simulink model "microgrid_case5"  (R2026a)
settings: Solver=ode14x  FixedStep=50e-6
libraries: ee_lib x65, nesl_utility x33, fl_lib x29, simulink x2
(part 2 of 2)

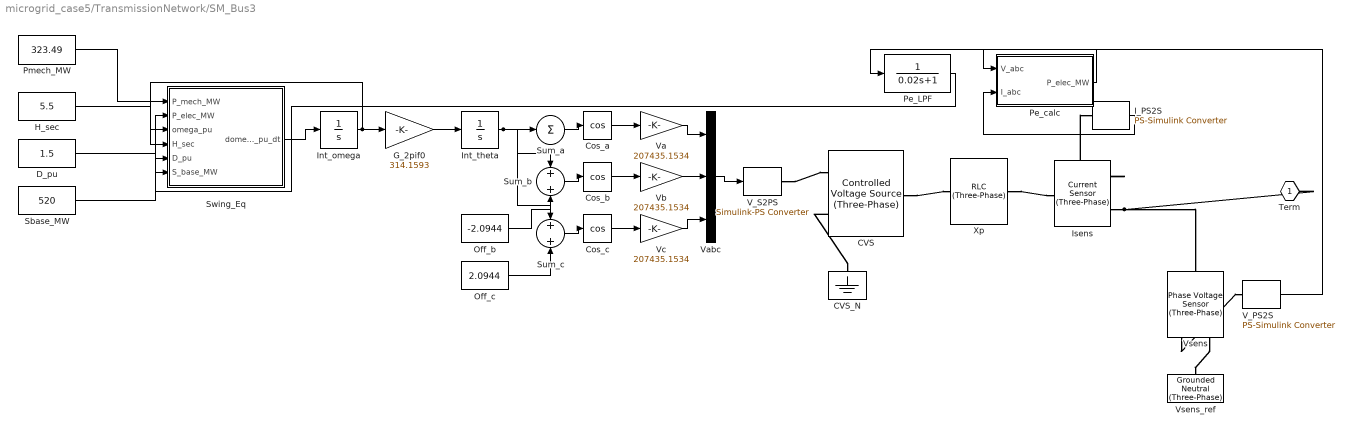
== system microgrid_case5/TransmissionNetwork/SM_Bus3 ==
  CVS : ee_lib/Sources/Controlled Voltage Source (Three-Phase)  input_option=ee.enum.inputType.instantaneous  FRated=60 Hz
  CVS_N : fl_lib/Electrical/Electrical Elements/Electrical Reference
  Cos_a : Trigonometry  Operator=cos
  Cos_b : Trigonometry  Operator=cos
  Cos_c : Trigonometry  Operator=cos
  D_pu : Constant  Value=1.5
  G_2pif0 : Gain  Gain=314.1593
  H_sec : Constant  Value=5.5
  I_PS2S : nesl_utility/PS-Simulink Converter  PhysicalDomain=network_engine_domain  SubClassName=ps_output  LeftPortType=input  RightPortType=output  PseudoPeriodic=off  Frequencies=[]  VectorFormat=inherit  Unit=inherit  AffineConversion=off
  Int_omega : Integrator  InitialCondition=1.0
  Int_theta : Integrator  InitialCondition=0.13268
  Isens : ee_lib/Sensors & Transducers/Current Sensor (Three-Phase)  port_option=ee.enum.threePhasePort.composite
  Off_b : Constant  Value=-2.0944
  Off_c : Constant  Value=2.0944
  Pe_LPF : TransferFcn  Denominator=[0.02 1]
  Pe_calc : MATLAB Function  TreatAsAtomicUnit=on
  Pmech_MW : Constant  Value=323.49
  Sbase_MW : Constant  Value=520
  Sum_a : Sum  Inputs=+
  Sum_b : Sum
  Sum_c : Sum
  Swing_Eq : MATLAB Function  TreatAsAtomicUnit=on
  V_PS2S : nesl_utility/PS-Simulink Converter  PhysicalDomain=network_engine_domain  SubClassName=ps_output  LeftPortType=input  RightPortType=output  PseudoPeriodic=off  Frequencies=[]  VectorFormat=inherit  Unit=inherit  AffineConversion=off
  V_S2PS : nesl_utility/Simulink-PS Converter  PhysicalDomain=network_engine_domain  SubClassName=ps_input  LeftPortType=input  RightPortType=output  PseudoPeriodic=off  Frequencies=[]  NoiseDistribution=none  NoiseParameters=[]  Unit=V  AffineConversion=off  FilteringAndDerivatives=filter  SimscapeFilterOrder=1  InputFilterTimeConstant=1e-4  UdotUserProvided=0
  Va : Gain  Gain=207435.1534
  Vabc : Mux  Inputs=3
  Vb : Gain  Gain=207435.1534
  Vc : Gain  Gain=207435.1534
  Vsens : ee_lib/Sensors & Transducers/Phase Voltage Sensor (Three-Phase)  port_option=ee.enum.threePhasePort.composite
  Vsens_ref : ee_lib/Connectors & References/Grounded Neutral (Three-Phase)  port_option=ee.enum.threePhasePort.composite
  Xp : ee_lib/Passive/RLC Assemblies/RLC (Three-Phase)  port_option=ee.enum.threePhasePort.composite  component_structure=ee.enum.rlc.structure.SeriesRL  R=0.001 Ohm  L=0.080955 H  C=1e-6 F  R_parasitic=0 Ohm  G_parasitic=0 1/Ohm  IL_specify=off  IL_priority=High  IL=[0, 0, 0] A  IL_nominal_specify=off  IL_nominal_value=1  IL_nominal_unit=A  VC_specify=off  VC_priority=High  VC=[0, 0, 0] V  VC_nominal_specify=off  VC_nominal_value=1  VC_nominal_unit=V
  Term : PMIOPort  Side=Right
  wires:
  V_PS2S/1 -> Pe_calc/1(V_abc)
  I_PS2S/1 -> Pe_calc/2(I_abc)
  Pe_calc/1(P_elec_MW) -> Pe_LPF/1
  Pmech_MW/1 -> Swing_Eq/1(P_mech_MW)
  Pe_LPF/1 -> Swing_Eq/2(P_elec_MW)
  Int_omega/1 -> Swing_Eq/3(omega_pu), G_2pif0/1
  H_sec/1 -> Swing_Eq/4(H_sec)
  D_pu/1 -> Swing_Eq/5(D_pu)
  Sbase_MW/1 -> Swing_Eq/6(S_base_MW)
  Swing_Eq/1(domega_pu_dt) -> Int_omega/1
  G_2pif0/1 -> Int_theta/1
  Int_theta/1 -> Sum_a/1, Sum_b/1, Sum_c/1
  Off_b/1 -> Sum_b/2
  Off_c/1 -> Sum_c/2
  Sum_a/1 -> Cos_a/1
  Sum_b/1 -> Cos_b/1
  Sum_c/1 -> Cos_c/1
  Cos_a/1 -> Va/1
  Cos_b/1 -> Vb/1
  Cos_c/1 -> Vc/1
  Va/1 -> Vabc/1
  Vb/1 -> Vabc/2
  Vc/1 -> Vabc/3
  Vabc/1 -> V_S2PS/1
  connections:
  CVS/LConn2 -- CVS_N/LConn1
  V_S2PS/RConn1 -- CVS/LConn1
  CVS/RConn1 -- Xp/LConn1
  Xp/RConn1 -- Isens/LConn1
  Term/RConn1 -- Isens/RConn2 -- Vsens/LConn1
  Vsens/RConn2 -- Vsens_ref/LConn1
  Isens/RConn1 -- I_PS2S/LConn1
  Vsens/RConn1 -- V_PS2S/LConn1

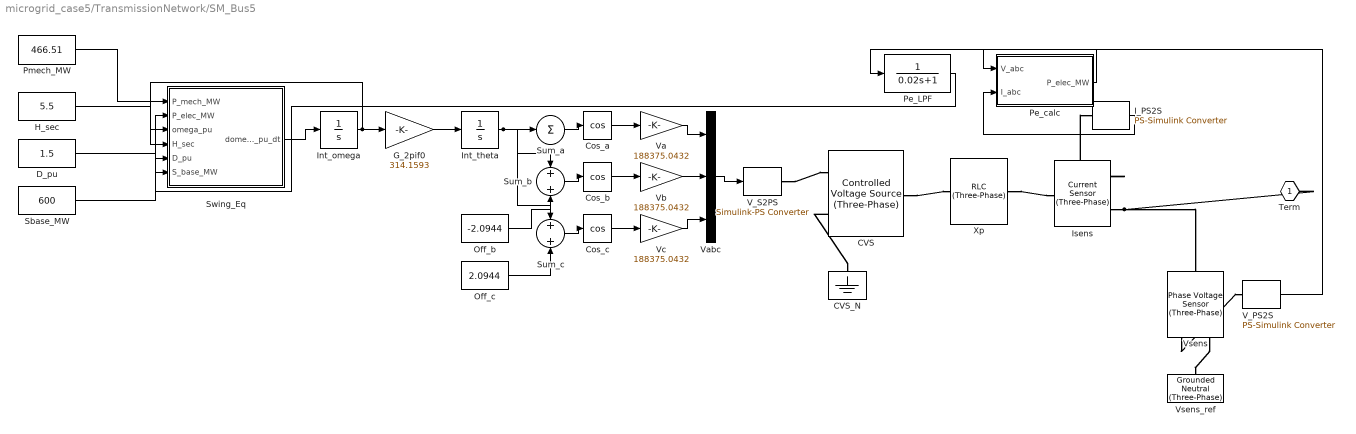
== system microgrid_case5/TransmissionNetwork/SM_Bus5 ==
  CVS : ee_lib/Sources/Controlled Voltage Source (Three-Phase)  input_option=ee.enum.inputType.instantaneous  FRated=60 Hz
  CVS_N : fl_lib/Electrical/Electrical Elements/Electrical Reference
  Cos_a : Trigonometry  Operator=cos
  Cos_b : Trigonometry  Operator=cos
  Cos_c : Trigonometry  Operator=cos
  D_pu : Constant  Value=1.5
  G_2pif0 : Gain  Gain=314.1593
  H_sec : Constant  Value=5.5
  I_PS2S : nesl_utility/PS-Simulink Converter  PhysicalDomain=network_engine_domain  SubClassName=ps_output  LeftPortType=input  RightPortType=output  PseudoPeriodic=off  Frequencies=[]  VectorFormat=inherit  Unit=inherit  AffineConversion=off
  Int_omega : Integrator  InitialCondition=1.0
  Int_theta : Integrator  InitialCondition=0.26678
  Isens : ee_lib/Sensors & Transducers/Current Sensor (Three-Phase)  port_option=ee.enum.threePhasePort.composite
  Off_b : Constant  Value=-2.0944
  Off_c : Constant  Value=2.0944
  Pe_LPF : TransferFcn  Denominator=[0.02 1]
  Pe_calc : MATLAB Function  TreatAsAtomicUnit=on
  Pmech_MW : Constant  Value=466.51
  Sbase_MW : Constant  Value=600
  Sum_a : Sum  Inputs=+
  Sum_b : Sum
  Sum_c : Sum
  Swing_Eq : MATLAB Function  TreatAsAtomicUnit=on
  V_PS2S : nesl_utility/PS-Simulink Converter  PhysicalDomain=network_engine_domain  SubClassName=ps_output  LeftPortType=input  RightPortType=output  PseudoPeriodic=off  Frequencies=[]  VectorFormat=inherit  Unit=inherit  AffineConversion=off
  V_S2PS : nesl_utility/Simulink-PS Converter  PhysicalDomain=network_engine_domain  SubClassName=ps_input  LeftPortType=input  RightPortType=output  PseudoPeriodic=off  Frequencies=[]  NoiseDistribution=none  NoiseParameters=[]  Unit=V  AffineConversion=off  FilteringAndDerivatives=filter  SimscapeFilterOrder=1  InputFilterTimeConstant=1e-4  UdotUserProvided=0
  Va : Gain  Gain=188375.0432
  Vabc : Mux  Inputs=3
  Vb : Gain  Gain=188375.0432
  Vc : Gain  Gain=188375.0432
  Vsens : ee_lib/Sensors & Transducers/Phase Voltage Sensor (Three-Phase)  port_option=ee.enum.threePhasePort.composite
  Vsens_ref : ee_lib/Connectors & References/Grounded Neutral (Three-Phase)  port_option=ee.enum.threePhasePort.composite
  Xp : ee_lib/Passive/RLC Assemblies/RLC (Three-Phase)  port_option=ee.enum.threePhasePort.composite  component_structure=ee.enum.rlc.structure.SeriesRL  R=0.001 Ohm  L=0.070161 H  C=1e-6 F  R_parasitic=0 Ohm  G_parasitic=0 1/Ohm  IL_specify=off  IL_priority=High  IL=[0, 0, 0] A  IL_nominal_specify=off  IL_nominal_value=1  IL_nominal_unit=A  VC_specify=off  VC_priority=High  VC=[0, 0, 0] V  VC_nominal_specify=off  VC_nominal_value=1  VC_nominal_unit=V
  Term : PMIOPort  Side=Right
  wires:
  V_PS2S/1 -> Pe_calc/1(V_abc)
  I_PS2S/1 -> Pe_calc/2(I_abc)
  Pe_calc/1(P_elec_MW) -> Pe_LPF/1
  Pmech_MW/1 -> Swing_Eq/1(P_mech_MW)
  Pe_LPF/1 -> Swing_Eq/2(P_elec_MW)
  Int_omega/1 -> Swing_Eq/3(omega_pu), G_2pif0/1
  H_sec/1 -> Swing_Eq/4(H_sec)
  D_pu/1 -> Swing_Eq/5(D_pu)
  Sbase_MW/1 -> Swing_Eq/6(S_base_MW)
  Swing_Eq/1(domega_pu_dt) -> Int_omega/1
  G_2pif0/1 -> Int_theta/1
  Int_theta/1 -> Sum_a/1, Sum_b/1, Sum_c/1
  Off_b/1 -> Sum_b/2
  Off_c/1 -> Sum_c/2
  Sum_a/1 -> Cos_a/1
  Sum_b/1 -> Cos_b/1
  Sum_c/1 -> Cos_c/1
  Cos_a/1 -> Va/1
  Cos_b/1 -> Vb/1
  Cos_c/1 -> Vc/1
  Va/1 -> Vabc/1
  Vb/1 -> Vabc/2
  Vc/1 -> Vabc/3
  Vabc/1 -> V_S2PS/1
  connections:
  CVS/LConn2 -- CVS_N/LConn1
  V_S2PS/RConn1 -- CVS/LConn1
  CVS/RConn1 -- Xp/LConn1
  Xp/RConn1 -- Isens/LConn1
  Term/RConn1 -- Isens/RConn2 -- Vsens/LConn1
  Vsens/RConn2 -- Vsens_ref/LConn1
  Isens/RConn1 -- I_PS2S/LConn1
  Vsens/RConn1 -- V_PS2S/LConn1

== matlab function microgrid_case5/TransmissionNetwork/SM_Bus5/Pe_calc ==
  data: V_abc input; P_elec_MW output; I_abc input
function P_elec_MW = Pe_calc(V_abc, I_abc)
%#codegen
% Instantaneous 3-phase electrical power at the machine terminal [MW].
    P_W       = V_abc(1)*I_abc(1) + V_abc(2)*I_abc(2) + V_abc(3)*I_abc(3);
    P_elec_MW = P_W / 1e6;
end

== matlab function microgrid_case5/PCC/PLL_freq ==
  settings: updateMethod=DISCRETE  sampleTime=5e-05
  data: v_abc input; f_meas_Hz output; dt_s input; f0_Hz input; Kp input; Ki input
function f_meas_Hz = PLL_freq(v_abc, dt_s, f0_Hz, Kp, Ki)
%#codegen
% Synchronous-reference-frame PLL on the MV phase voltages.
% Clarke (amplitude-invariant) → normalise → q-axis error → PI → θ.
% Persistent θ and integral are discrete states (HIL/codegen friendly).
    persistent th vi
    if isempty(th), th = 0; vi = 0; end
    va = v_abc(1); vb = v_abc(2); vc = v_abc(3);
    valpha = (2/3)*(va - 0.5*vb - 0.5*vc);
    vbeta  = (1/sqrt(3))*(vb - vc);
    Vm = hypot(valpha, vbeta) + 1e-9;       % avoid /0 at start-up
    sa = valpha/Vm; sb = vbeta/Vm;          % unit phasor (amplitude-independent)
    vq = -sa*sin(th) + sb*cos(th);          % q-axis error → 0 when locked
    vi = vi + Ki*vq*dt_s;                    % PI integral
    w  = 2*pi*f0_Hz + Kp*vq + vi;            % estimated angular frequency
    th = mod(th + w*dt_s, 2*pi);             % advance & wrap phase
    f_meas_Hz = w/(2*pi);
end

== matlab function microgrid_case5/PCC/V_to_pu ==
  data: v_abc input; V_pcc_pu output; Vbase_LL input
function V_pcc_pu = V_to_pu(v_abc, Vbase_LL)
%#codegen
% Line-to-line RMS per-unit from instantaneous phase voltages.
% Amplitude-invariant Clarke magnitude = peak phase amplitude;
% LL_RMS = peak_phase * sqrt(3)/sqrt(2)  →  pu = LL_RMS / Vbase_LL.
    va = v_abc(1); vb = v_abc(2); vc = v_abc(3);
    valpha = (2/3)*(va - 0.5*vb - 0.5*vc);
    vbeta  = (1/sqrt(3))*(vb - vc);
    Vphase_peak = hypot(valpha, vbeta);
    V_pcc_pu = Vphase_peak * sqrt(3/2) / Vbase_LL;
end

== matlab function microgrid_case5/PCC/PQ_calc ==
  data: v_abc input; P_MW output; i_abc input; Q_MVAr output
function [P_MW, Q_MVAr] = PQ_calc(v_abc, i_abc)
%#codegen
% Instantaneous three-phase active & reactive power at the MV node.
% Amplitude-invariant Clarke → P = 1.5(vα iα + vβ iβ),  Q = 1.5(vβ iα − vα iβ).
% Sign: + current is transmission→MG, so +P = MG importing (§1.1).
    va = v_abc(1); vb = v_abc(2); vc = v_abc(3);
    ia = i_abc(1); ib = i_abc(2); ic = i_abc(3);
    valpha = (2/3)*(va - 0.5*vb - 0.5*vc);  vbeta = (1/sqrt(3))*(vb - vc);
    ialpha = (2/3)*(ia - 0.5*ib - 0.5*ic);  ibeta = (1/sqrt(3))*(ib - ic);
    P_W   = 1.5*(valpha*ialpha + vbeta*ibeta);
    Q_VAR = 1.5*(vbeta*ialpha - valpha*ibeta);
    P_MW   = P_W   / 1e6;
    Q_MVAr = Q_VAR / 1e6;
end

== matlab function microgrid_case5/GridFormingVSC/vf_droop ==
  settings: updateMethod=DISCRETE  sampleTime=5e-05
  data: v_abc input; m_abc output; i_abc input; V_dc_V input; f_meas_Hz input; V_meas_pu input; V_ref_pu input; f_ref_Hz input; mode input; dt_s input; f0_Hz input; CB_grid input; f_cmd_Hz output; P_vsc_MW output; Q_vsc_MVAr output; cb_open output; i_d_A output; i_q_A output; i_d_ref_A output; i_q_ref_A output
function [m_abc, f_cmd_Hz, P_vsc_MW, Q_vsc_MVAr, cb_open, i_d_A, i_q_A, i_d_ref_A, i_q_ref_A] = vf_droop(v_abc, i_abc, V_dc_V, f_meas_Hz, V_meas_pu, V_ref_pu, f_ref_Hz, mode, dt_s, f0_Hz, CB_grid)
%#codegen
% Grid-forming V-f droop + A8 secondary restoration (IO_CONTRACTS §3.5).
% FAZ 1+2 (2026-07-04, G10): optional inner dq current loop, gated by
% inner_en below. Default inner_en=0 reproduces the legacy open-loop m
% synthesis EXACTLY (bit-for-bit bypass).
% Persistent discrete states: oscillator phase, P/Q filters, secondary
% integrators, soft-start clock, saturation flag, inner current-loop PIs.
S_base_VA = 350000000;    % droop power base = VSC rating
R_p   = 0.05;  R_q   = 0.05;   % droop SLOPES (G4: §3.5 "(1/R)" read as slope)
tauPQ = 0.01;                  % P/Q LPF [s] (G5)
Kp_f  = 0.1;  Ki_f  = 0.5;  df_max = 2.5;  % A8 f-restore + clamp
Kp_V  = 0.5;  Ki_V  = 2;  dV_max = 0.1;  % A8 V-restore + clamp
Vph_pk = 563.383;  Vdc_nom = 1500;  m_lim = 1;
t_soft = 0.2;                 % amplitude ramp [s] (G3)
t_blend = 0.1;                % post-close amplitude blend [s] (G8)
Kdc_WpV = 3.33333e+06;  P_exp_max_W = 1e+08;  % DC-link export droop (A)
Kp_i = 3.11143;  Ki_i = 39.0994;  % FAZ1+2 inner current PI (33kV side, G10)
L_c = 0.000990398;  R_c = 0.0124457;  % coupling L[H]/R[Ohm] = XFMR leakage (G1), no separate filter
n_t = 47.8261;  % step-up XFMR turns ratio MV/LV (G10a init fix): AVVSC=LV, sensing=MV
i_max_pk = 9525.79;  % current limit, PEAK amps (id/iq are peak-scale, amplitude-invariant)
ilim_exit = 0.95*i_max_pk;  t_ib = 0.005;  % FAZ3 (G10b) limit hysteresis-lo + exit blend [s]
inner_en = 1;  % FAZ3 enable: 0=pure legacy voltage-forming, 1=overcurrent current-limiter armed
    persistent th P_f Q_f int_f int_V t_run sat_prev cb_state t_close id_int iq_int inner_prev ilim_on w_blend
    if isempty(th)
        % G8: start the LV oscillator ON the measured bus phase so the
        % pre-sync pull converges fast (Yg/D11: MV leads LV +30°).
        th = atan2((1/sqrt(3))*(v_abc(2)-v_abc(3)), ...
                   (2/3)*(v_abc(1)-0.5*v_abc(2)-0.5*v_abc(3))) - pi/6;
        P_f=0; Q_f=0; int_f=0; int_V=0; t_run=0; sat_prev=0;
        cb_state=0; t_close=0;              % G8: sync breaker starts OPEN
        id_int=0; iq_int=0; inner_prev=0;   % FAZ1+2: inner current-loop PI states + edge flag (G10a)
        ilim_on=0; w_blend=0;               % FAZ3 (G10b): overcurrent latch + legacy<->inner blend weight
    end

    % ── Instantaneous P/Q at the 33 kV terminal (amplitude-invariant Clarke)
    va=v_abc(1); vb=v_abc(2); vc=v_abc(3); ia=i_abc(1); ib=i_abc(2); ic=i_abc(3);
    valpha=(2/3)*(va-0.5*vb-0.5*vc);  vbeta=(1/sqrt(3))*(vb-vc);
    ialpha=(2/3)*(ia-0.5*ib-0.5*ic);  ibeta=(1/sqrt(3))*(ib-ic);
    P_W   = 1.5*(valpha*ialpha + vbeta*ibeta);   % + = injecting into AC bus
    Q_VAR = 1.5*(vbeta*ialpha - valpha*ibeta);
    P_f = P_f + (P_W   - P_f)*dt_s/tauPQ;        % 1st-order measurement LPF
    Q_f = Q_f + (Q_VAR - Q_f)*dt_s/tauPQ;
    Vdc_eff = max(V_dc_V, 0.5*Vdc_nom);          % FAZ1+2: moved up, needed before the oscillator section

    % ── Soft-start amplitude ramp (G3); integrators frozen until the
    % sync breaker is closed AND the post-close blend is done (G8).
    t_run = t_run + dt_s;
    soft  = min(t_run/t_soft, 1);
    conn  = (cb_state > 0.5) && (t_run - t_close >= t_blend);

    if mode > 0.5   % ─── GRID-FORMING (A2: no anti-islanding delay) ───
        % A8 secondary restoration: slow PIs trim f_ref/V_ref so the
        % steady state returns to the setpoints despite the droop offset.
        err_f = f_ref_Hz - f_meas_Hz;
        err_V = V_ref_pu - V_meas_pu;
        % Rule 7 anti-windup: integrate only when the modulator was NOT
        % saturated last step and the unit is CONNECTED + blended (G8).
        if sat_prev < 0.5 && conn
            int_f = int_f + Ki_f*err_f*dt_s;
            int_V = int_V + Ki_V*err_V*dt_s;
        end
        int_f = max(-df_max, min(df_max, int_f));    % clamp (Rule 7)
        int_V = max(-dV_max, min(dV_max, int_V));
        df_restore = max(-df_max, min(df_max, Kp_f*err_f + int_f));
        dV_restore = max(-dV_max, min(dV_max, Kp_V*err_V + int_V));

        % DC-LINK VOLTAGE DROOP (A): export DC-bus surplus to the grid. When
        % V_dc rises above nominal (ESS saturated on surplus renewables), bias
        % the droop frequency UP so the VSC angle leads the grid and real power
        % flows OUT, pulling V_dc back. df_export = R_p*f0*(P_export/S) makes the
        % converter settle at P=P_export (steady state f_cmd=grid f). Grid-
        % connected ONLY (CB_grid) AND synced (conn); island has no grid → 0.
        df_export = 0;
        if CB_grid > 0.5 && conn
            P_exp_W = Kdc_WpV*(V_dc_V - Vdc_nom);
            if P_exp_W < 0, P_exp_W = 0; end
            if P_exp_W > P_exp_max_W, P_exp_W = P_exp_max_W; end
            df_export = R_p*f0_Hz*(P_exp_W/S_base_VA);
        end
        % PRIMARY droop (slope form, G4): rated P → R_p·f0 Hz sag.
        f_cmd_Hz = (f_ref_Hz + df_restore + df_export) - R_p*(P_f/S_base_VA)*f0_Hz;
        V_cmd_pu = (V_ref_pu + dV_restore) - R_q*(Q_f/S_base_VA);
    else            % ─── GRID-FOLLOWING (stub, G7) ───
        f_cmd_Hz = f_meas_Hz;        % track the grid; droop/secondary off
        V_cmd_pu = V_ref_pu;
    end

    % ══════════════════════════════════════════════════════════════════
    % FAZ 1+2 (G10) — INNER dq CURRENT LOOP, island/grid-forming path only.
    % Yazdani & Iravani 2010 cascaded VSC control. th used below is THIS
    % sample angle (BEFORE the oscillator update further down) — the same
    % instant the v_abc/i_abc measurements were taken.
    % ══════════════════════════════════════════════════════════════════
    c_th = cos(th); s_th = sin(th);
    i_d_A = ialpha*c_th + ibeta*s_th;   % Park (amplitude-invariant -> PEAK
    i_q_A = -ialpha*s_th + ibeta*c_th;  % scale, matches i_abc directly, NOT rms)
    % ══ FAZ 3 (G10b): GRID-FORMING with CURRENT LIMITING (Rocabert 2012). The
    % VSC stays VOLTAGE-forming (m_abc_legacy forms f) in NORMAL operation; the
    % inner dq loop engages ONLY on OVERCURRENT, as a current LIMITER. It is NOT
    % an always-on current source (that let nobody form f -> f drifted to 53.76
    % Hz). Hysteresis latch: enter at i_max, leave below ilim_exit (0.95*i_max).
    i_mag = sqrt(i_d_A*i_d_A + i_q_A*i_q_A);
    if i_mag > i_max_pk,  ilim_on = 1; end   % over-limit -> arm the limiter
    if i_mag < ilim_exit, ilim_on = 0; end   % recovered  -> release (hysteresis)
    inner_active = double((mode > 0.5) && (inner_en > 0.5) && conn && (ilim_on > 0.5));
    % Output blend weight w_blend: jumps to 1 while limiting (the G10a bumpless
    % preload keeps the ENTRY step-free), decays to 0 over t_ib on release (soft
    % handback to legacy voltage-forming). inner_compute keeps the inner PI/phasor
    % coherent through the decay window so the blend has a live target.
    if inner_active > 0.5
        w_blend = 1;
    else
        w_blend = max(0, w_blend - dt_s/t_ib);
    end
    inner_compute = (inner_active > 0.5) || (w_blend > 1e-3);
    if inner_compute
        v_d = valpha*c_th + vbeta*s_th;
        v_q = -valpha*s_th + vbeta*c_th;
        % FAZ 3 current reference = the MEASURED current direction clamped onto
        % the i_max_pk circle. Over-limit: scl<1 pulls |i| down to i_max (id/iq
        % share preserved -- the protective action). Blend-out (not over-limit):
        % scl=1 = identity -> the inner voltage tracks the present operating
        % point and converges to legacy, so the handback is smooth.
        if inner_active > 0.5 && i_mag > 1e-6
            scl = i_max_pk / i_mag;
        else
            scl = 1;
        end
        i_d_ref_A = i_d_A * scl;
        i_q_ref_A = i_q_A * scl;
        % Decoupled PI (Yazdani & Iravani form).
        e_id = i_d_ref_A - i_d_A;  e_iq = i_q_ref_A - i_q_A;
        omega_c = 2*pi*f_meas_Hz;
        if inner_active > 0.5 && inner_prev < 0.5
            % G10a BUMPLESS TRANSFER at the RISING edge of current-limiting:
            % preload integrators so vd_star/vq_star equal the LEGACY converter
            % voltage this very step -- d = n_t*V_cmd_pu*Vph_pk (MV-referred),
            % q = 0 -- making m_abc_inner == m_abc_legacy at the handoff (no
            % voltage step across the leakage inductance).
            id_int = n_t*V_cmd_pu*Vph_pk - v_d + omega_c*L_c*i_q_A - Kp_i*e_id;
            iq_int = -v_q - omega_c*L_c*i_d_A - Kp_i*e_iq;
        elseif inner_active > 0.5
            % actively limiting: integrate (circle reference is always feasible,
            % and limiting lowers m -> no ceiling windup, Rule 7 satisfied).
            id_int = id_int + Ki_i*e_id*dt_s;
            iq_int = iq_int + Ki_i*e_iq*dt_s;
        end
        % (blend-out: integrators FROZEN at their release value; identity ref
        %  gives e~0 so vd_star holds a coherent phasor that decays into legacy.)
        vd_star = v_d - omega_c*L_c*i_q_A + Kp_i*e_id + id_int;
        vq_star = v_q + omega_c*L_c*i_d_A + Kp_i*e_iq + iq_int;
        valpha_s = vd_star*c_th - vq_star*s_th;   % inverse Park
        vbeta_s  = vd_star*s_th + vq_star*c_th;
        % G10a: /n_t refers the MV-side command back through the step-up
        % transformer to the LV converter terminal before m = 2*v_conv/Vdc.
        m_abc_inner = (2/(n_t*Vdc_eff)) * [ valpha_s; ...                   % inverse Clarke
                                      -0.5*valpha_s + (sqrt(3)/2)*vbeta_s; ...
                                      -0.5*valpha_s - (sqrt(3)/2)*vbeta_s ];
    else
        i_d_ref_A = 0;  i_q_ref_A = 0;  m_abc_inner = [0;0;0];
    end
    inner_prev = double(inner_active);   % G10a/b: rising-edge tracker for the bumpless preload

    % ── Oscillator + modulation wave.  v_phase = m·V_dc/2 (verified), so
    % m = V_target_pk/(V_dc/2) with MEASURED V_dc (G6 backstop: V_dc sag
    % → m ceiling → AC sags too; no energy from nothing).
    % ── G8 SYNC BREAKER + pre-sync state machine. Behind the OPEN
    % breaker the converter only magnetizes its own unloaded step-up,
    % so the t=0 m=0 instant cannot bolt a fault on the live bus. The
    % bus-side sensors keep reading the live grid: ramp the unloaded LV
    % to the measured |V| while k_sync locks th to (φ_bus − 30°), then
    % CLOSE on phase match and blend amplitude to the droop command.
    k_sync  = 30;                            % phase pull gain [1/s]
    phi_bus = atan2(vbeta, valpha);
    e_th    = atan2(sin(phi_bus - pi/6 - th), cos(phi_bus - pi/6 - th));
    if cb_state < 0.5                        % ── OPEN: pre-synchronize
        % dead-bus close needs t_run>0.05 s: the V_pcc measurement reads
        % ~0 for the first samples (discrete startup), which must not be
        % mistaken for a dead bus (it closed the breaker at 100 us once).
        if V_meas_pu < 0.05 && t_run > 0.05
            cb_state = 1;  t_close = t_run;  % dead bus: black start
        elseif soft >= 1 && abs(e_th) < 0.03
            cb_state = 1;  t_close = t_run;  % matched: connect
        end
        th    = th + (2*pi*f_cmd_Hz + k_sync*e_th)*dt_s;
        V_eff = soft * V_meas_pu;            % land on the bus magnitude
    else                                     % ── CLOSED
        th = th + 2*pi*f_cmd_Hz*dt_s;
        if V_meas_pu > 0.05
            mu    = min((t_run - t_close)/t_blend, 1);
            V_eff = (1-mu)*V_meas_pu + mu*V_cmd_pu;  % soft handoff
        else
            V_eff = soft * V_cmd_pu;         % black start: plain G3 ramp
        end
    end
    th = mod(th, 2*pi);
    m_pk = V_eff * Vph_pk / (Vdc_eff/2);
    if m_pk > m_lim
        m_pk = m_lim;  sat_prev = 1;     % freeze integrators next step
    else
        sat_prev = 0;
    end
    m_abc_legacy = m_pk * [cos(th); cos(th - 2*pi/3); cos(th + 2*pi/3)];

    % FAZ 3 selection (G10b): blend legacy voltage-forming <-> inner current-
    % limiter by w_blend. w_blend=0 (normal, no overcurrent) -> PURE legacy so
    % the VSC forms f; w_blend=1 (limiting) -> pure inner so |i| is clamped to
    % i_max; the decay is the soft handback. inner_en=0 keeps ilim_on/w_blend at
    % 0 -> legacy only, bit-for-bit bypass preserved.
    m_sel = (1 - w_blend)*m_abc_legacy + w_blend*m_abc_inner;
    m_abc = max(-m_lim, min(m_lim, m_sel));

    P_vsc_MW   = P_f/1e6;                % filtered, + = injecting (§1.1)
    Q_vsc_MVAr = Q_f/1e6;
    cb_open    = 1 - cb_state;           % G8: breaker ctrl (>0.5 = OPEN)
end

== matlab function microgrid_case5/PV/pv_cell ==
  settings: updateMethod=DISCRETE  sampleTime=5e-05
  data: V_op input; I_pv output; G input; T_amb input; P_panel_W output
function [I_pv, P_panel_W] = pv_cell(V_op, G, T_amb)
%#codegen
% Single-diode array (INLINE twin of PARAMS/pv_iv.m). One equivalent array.
Voc_stc = 900;  N_s = 1500;  nID = 1.3;
Isc_stc = 132188;  aIsc = 0.0005;  bVoc = -0.004;  NOCT = 45;
    q = 1.602176634e-19;  kB = 1.380649e-23;
    Tcell = T_amb + (NOCT - 20)/800 * G;
    a  = N_s * nID * kB * (Tcell + 273.15) / q;
    Iph = (G/1000) * Isc_stc * (1 + aIsc*(Tcell - 25));
    if Iph <= 0
        I_pv = 0; P_panel_W = 0; return;
    end
    Voc_T = Voc_stc * (1 + bVoc*(Tcell - 25));
    I0 = Iph / (exp(Voc_T/a) - 1);
    I_pv = Iph - I0*(exp(V_op/a) - 1);
    if I_pv < 0, I_pv = 0; end
    P_panel_W = V_op * I_pv;
end

== matlab function microgrid_case5/PV/mppt_po ==
  settings: updateMethod=DISCRETE  sampleTime=5e-05
  data: P_meas input; V_ref output; dt input
function V_ref = mppt_po(P_meas, dt)
%#codegen
% Perturb & Observe MPPT. Perturbs every ~1 ms; climbs the P(V) hill.
Vinit = 702;  dV = 2;  Vmin = 50;  Vmax = 900;  period = 1e-3;
    persistent Vr Pp dir cnt
    if isempty(Vr), Vr = Vinit; Pp = 0; dir = 1; cnt = 0; end
    nper = round(period/dt);
    cnt = cnt + 1;
    if cnt >= nper
        if P_meas < Pp, dir = -dir; end     % got worse → reverse direction
        Vr = Vr + dir*dV;
        if Vr > Vmax, Vr = Vmax; end
        if Vr < Vmin, Vr = Vmin; end
        Pp = P_meas;
        cnt = 0;
    end
    V_ref = Vr;
end

== matlab function microgrid_case5/PV/dcdc_ctrl ==
  settings: updateMethod=DISCRETE  sampleTime=5e-05
  data: P_panel_W input; I_cmd_A output; V_dc_V input; P_bus_MW output
function [I_cmd_A, P_bus_MW] = dcdc_ctrl(P_panel_W, V_dc_V)
%#codegen
% Averaged boost: deliver P_panel·η to the bus as a current I = P_bus/V_dc.
eta = 0.784;  Vfloor = 750;
    P_bus_W  = P_panel_W * eta;
    I_cmd_A  = P_bus_W / max(V_dc_V, Vfloor);
    P_bus_MW = P_bus_W / 1e6;
end

== matlab function microgrid_case5/Wind/wind_turbine ==
  settings: updateMethod=DISCRETE  sampleTime=5e-05
  data: v input; P_turb_W output; Cp output
function [P_turb_W, Cp] = wind_turbine(v)
%#codegen
% Four-region curve. Cube region runs at Cp_max (optimal λ, β=0); above
% v_rated the turbine pitches (P held at P_rated, effective Cp falls).
Cpmax = 0.480012;  rho = 1.225;  A = 408153.32;
cin = 3;  vr = 10;  cout = 25;  Prated = 1.2e+08;
    if v < cin || v >= cout
        P_turb_W = 0; Cp = 0; return;     % below cut-in or past cut-out
    end
    Pwind = 0.5*rho*A*v^3;                % power in the wind through area A
    Pmech = Cpmax * Pwind;                % cube region at optimal lambda
    if Pmech > Prated
        P_turb_W = Prated;                % pitch-regulated plateau
        Cp = Prated / Pwind;              % effective Cp (< Cp_max)
    else
        P_turb_W = Pmech;                 % cube region
        Cp = Cpmax;
    end
end

== matlab function microgrid_case5/Wind/dcdc_ctrl ==
  settings: updateMethod=DISCRETE  sampleTime=5e-05
  data: P_turb_W input; I_cmd_A output; V_dc_V input; P_bus_MW output
function [I_cmd_A, P_bus_MW] = dcdc_ctrl(P_turb_W, V_dc_V)
%#codegen
% Averaged generator+rectifier+DC-DC: deliver P_turb·η to the bus as I=P/V.
eta = 0.855;  Vfloor = 750;
    P_bus_W  = P_turb_W * eta;
    I_cmd_A  = P_bus_W / max(V_dc_V, Vfloor);
    P_bus_MW = P_bus_W / 1e6;
end

== matlab function microgrid_case5/ESS/ess_ctrl ==
  settings: updateMethod=DISCRETE  sampleTime=5e-05
  data: V_dc_V input; I_cmd_A output; Pref_MW input; dt_s input; P_ess_MW output; SOC output; V_batt_V output
function [I_cmd_A, P_ess_MW, SOC, V_batt_V] = ess_ctrl(V_dc_V, Pref_MW, dt_s)
%#codegen
% ESS controller (IO_CONTRACTS §3.9): owns V_dc. slewed EMS feed-forward
% + unslewed PI trim (H7) -> TOTAL clamp (Rule 4, SOC-aware) -> CCS cmd.
% Signal-level Thevenin battery + SOC integrator (Rule 7 bounds).
V_set = 1500;     % DC bus setpoint [V]
Kp = 0.2;  Ki = 5;   % V_dc PI [MW/V], [MW/V/s] (H3)
Pmax = 80;  slew = 80;   % clamp [MW], slew [MW/s]
SOCmin = 0.15;  SOCmax = 0.9;  E_MWh = 200;
eta = 0.95;              % each-way efficiency (H5)
Voc0 = 700;  dVoc = 200;  Rint = 0.00016;
SOC0 = 0.6;
    persistent soc p_int pref_prev v_batt_prev sat_prev
    if isempty(soc)
        soc = SOC0; p_int = 0; pref_prev = 0;
        v_batt_prev = Voc0 + SOC0*dVoc; sat_prev = 0;
    end

    % ── V_dc PI trim (+ = inject power into the bus = discharge)
    err_V = V_set - V_dc_V;
    if sat_prev < 0.5                       % Rule 7: freeze while saturated
        p_int = p_int + Ki*err_V*dt_s;
    end
    p_int = max(-Pmax, min(Pmax, p_int));   % integral hard clamp

    % ── slew limit on the EMS dispatch FF ONLY (H7): slewing the PI trim
    % starves the 4.4 krad/s V_dc loop (4 kW/step) -> limit cycle.
    pref_slew = max(pref_prev - slew*dt_s, min(pref_prev + slew*dt_s, Pref_MW));
    pref_prev = pref_slew;
    P_sum = pref_slew + Kp*err_V + p_int;   % slewed FF + unslewed trim (H4/H7)

    % ── ONE total clamp (Rule 4) with SOC-aware directional limits
    P_hi = Pmax;  P_lo = -Pmax;
    if soc <= SOCmin, P_hi = 0; end         % empty: no more discharge
    if soc >= SOCmax, P_lo = 0; end         % full : no more charge
    P_act = max(P_lo, min(P_hi, P_sum));
    sat_prev = double(abs(P_act - P_sum) > 1e-9);   % clamp engaged

    % ── battery side (H5): discharge draws MORE than bus gets, charge
    % stores LESS than bus sends. SOC integrates the CELL power.
    if P_act >= 0, P_batt_MW = P_act/eta; else, P_batt_MW = P_act*eta; end
    soc = soc - P_batt_MW*dt_s/(3600*E_MWh);
    soc = max(SOCmin, min(SOCmax, soc));    % Rule 7 bounds

    % ── Thevenin diagnostic: V_batt = OCV(SOC) − R_int·I_batt.
    % Algebraic in V_batt → use previous-step V (fine at 50 µs).
    V_oc = Voc0 + soc*dVoc;
    I_batt = P_batt_MW*1e6 / max(v_batt_prev, 0.5*Voc0);
    V_batt_V = V_oc - Rint*I_batt;
    v_batt_prev = V_batt_V;

    % ── bus-side current command for the CCS (+ = inject into + rail)
    I_cmd_A = P_act*1e6 / max(V_dc_V, 750);
    P_ess_MW = P_act;
    SOC = soc;
end

== matlab function microgrid_case5/Electrolyzer/el_ctrl ==
  settings: updateMethod=DISCRETE  sampleTime=5e-05
  data: Pref_MW input; I_cmd_A output; V_dc_V input; dt_s input; P_elec_MW output; mdot_H2_kgs output; U_stack_V output
function [I_cmd_A, P_elec_MW, mdot_H2_kgs, U_stack_V] = el_ctrl(Pref_MW, V_dc_V, dt_s)
%#codegen
% PEM electrolyzer (Ulleberg polarization + Faraday). Draws power from the
% DC bus (LOAD: I_cmd < 0). See build_electrolyzer.m E1-E6.
N = 400;  A = 15;  T = 80;  Urev = 1.229;
Fc = 96485;  MH2 = 0.002016;  etaF = 0.99;  etaC = 0.97;
Pmax = 40;  Pmin = 5;  tau = 30;  slew = 13;  Vfloor = 750;
    persistent P_act P_ramp
    if isempty(P_act), P_act = 0; P_ramp = 0; end

    % ── command conditioning (Rule 4 single clamp): off, or [Pmin,Pmax]
    if Pref_MW < Pmin/2
        P_tgt = 0;                          % off (below half-min → shut down)
    else
        P_tgt = min(max(Pref_MW, Pmin), Pmax);
    end
    % ── slew the SETPOINT toward P_tgt (independent state), then lag the
    % realized power toward the slewed setpoint with the τ=30 s BoP lag (E4).
    % (P_ramp must NOT be tied to P_act, or the lag never sees the target.)
    dmax   = slew*dt_s;
    P_ramp = max(P_ramp - dmax, min(P_ramp + dmax, P_tgt));
    P_act  = P_act + (P_ramp - P_act)*dt_s/tau;
    P_elec_MW = P_act;

    % ── invert P_stack = N·U_cell(I)·I for the stack current (E2, bisection)
    P_stack = P_act*1e6*etaC;               % stack gets bus power · η_buck
    if P_stack < 1
        I = 0;  U_stack_V = N*Urev;          % off: open-circuit-ish
    else
        lo = 0;  hi = P_stack/(N*Urev);      % U_cell ≥ Urev → I ≤ this
        for it = 1:40
            mid = 0.5*(lo+hi);
            if N*electrolyzer_cell(mid/A, T)*mid < P_stack
                lo = mid;
            else
                hi = mid;
            end
        end
        I = 0.5*(lo+hi);
        U_stack_V = N*electrolyzer_cell(I/A, T);
    end

    % ── Faraday H2 production (E3, current-based, 2 e- per H2)
    mdot_H2_kgs = etaF * N * I / (2*Fc) * MH2;

    % ── bus-side current command: LOAD draws from +rail → NEGATIVE (E5)
    I_cmd_A = -P_act*1e6 / max(V_dc_V, Vfloor);
end

function U_cell = electrolyzer_cell(i, T)
%#codegen
% Ulleberg (2003) single-cell polarization. i = I/A [A/m^2], T [°C].
% U_cell = U_rev + ohmic(i,T) + activation(i,T).
    Urev = 1.229;                            % thermodynamic threshold [V]
    r1 = 8.05e-5;  r2 = -2.5e-7;             % ohmic   [Ω·m^2], [Ω·m^2/°C]
    s  = 0.185;                              % activation slope [V]
    t1 = -0.1002;  t2 = 8.424;  t3 = 247.3;  % activation [m^2/A], ·°C, ·°C^2
    r_ohm  = r1 + r2*T;
    t_coef = t1 + t2/T + t3/(T*T);
    arg = t_coef*i + 1;
    if arg < 1, arg = 1; end                 % keep log argument ≥ 1 (i ≥ 0)
    U_cell = Urev + r_ohm*i + s*log10(arg);
end

== matlab function microgrid_case5/PEMFC/fc_ctrl ==
  settings: updateMethod=DISCRETE  sampleTime=5e-05
  data: Pref_MW input; I_cmd_A output; V_dc_V input; dt_s input; P_fc_MW output; mdot_cons_kgs output; V_stack_V output
function [I_cmd_A, P_fc_MW, mdot_cons_kgs, V_stack_V] = fc_ctrl(Pref_MW, V_dc_V, dt_s)
%#codegen
% PEMFC (Correa polarization + Faraday consumption). SOURCES power to the DC
% bus (I_cmd > 0). See build_fc.m C1-C6.
Ns = 600;  K = 1.224e+08;  Fc = 96485;  MH2 = 0.002016;
etaU = 0.98;  etaC = 0.97;  Jhi = 1;
Pmax = 30;  Pmin = 2;  tau = 5;  slew = 12;  Vfloor = 750;
    persistent P_act P_ramp
    if isempty(P_act), P_act = 0; P_ramp = 0; end

    % ── command conditioning (Rule 4 single clamp): off, or [Pmin,Pmax]
    if Pref_MW < Pmin/2
        P_tgt = 0;
    else
        P_tgt = min(max(Pref_MW, Pmin), Pmax);
    end
    % ── independent slewed setpoint, then τ=5 s BoP lag (C4; EL bug lesson)
    dmax   = slew*dt_s;
    P_ramp = max(P_ramp - dmax, min(P_ramp + dmax, P_tgt));
    P_act  = P_act + (P_ramp - P_act)*dt_s/tau;
    P_fc_MW = P_act;

    % ── invert P_stack = K·V_cell(J)·J for J on the RISING branch (C2)
    P_stack = P_act*1e6/etaC;                % stack must make bus power / η_boost
    if P_stack < 1
        Jsol = 0;  mdot_cons_kgs = 0;
    else
        lo = 0;  hi = Jhi;
        for it = 1:40
            mid = 0.5*(lo+hi);
            if K*fc_cell(mid)*mid < P_stack
                lo = mid;
            else
                hi = mid;
            end
        end
        Jsol = 0.5*(lo+hi);
        Vc = fc_cell(Jsol);
        mdot_cons_kgs = (P_stack/Vc) * MH2 / (2*Fc*etaU);   % Faraday consumption (C3)
    end
    V_stack_V = Ns * fc_cell(max(Jsol, 1e-3));    % stack voltage (OCV-ish when off)

    % ── bus-side current command: SOURCE injects into +rail → POSITIVE (C5)
    I_cmd_A = P_act*1e6 / max(V_dc_V, Vfloor);
end

function V_cell = fc_cell(J)
%#codegen
% Correa et al. (2004) PEMFC single-cell polarization. J = current density
% [A/cm^2]. V_cell = E_nernst − V_act − V_ohm − V_con (DROPS with current).
    T = 75;  TK = T + 273.15;  A = 500;  pH2 = 1.5;  pO2 = 1.0;  Jmax = 1.5;
    x1 = -0.948;  x3 = 7.6e-5;  x4 = -1.93e-4;  B = 0.016;  RM = 0.00019;  RC = 0.00005;
    E = 1.229 - 0.85e-3*(TK-298.15) + 4.3085e-5*TK*(log(pH2) + 0.5*log(pO2));
    C_O2 = pO2/(5.08e6*exp(-498/TK));
    C_H2 = pH2/(1.09e6*exp(77/TK));
    x2 = 0.00286 + 0.0002*log(A) + 4.3e-5*log(C_H2);
    iFC = max(J*A, 1e-6);                          % per-cell current [A]
    Vact = -(x1 + x2*TK + x3*TK*log(C_O2) + x4*TK*log(iFC));   % activation loss
    Vohm = iFC*(RM + RC);                          % ohmic loss
    Vcon = -B*log(max(1 - J/Jmax, 1e-6));          % concentration loss
    V_cell = E - Vact - Vohm - Vcon;
end

== matlab function microgrid_case5/H2Tank/tank_dynamics ==
  settings: updateMethod=DISCRETE  sampleTime=5e-05
  data: mdot_prod_kgs input; m_H2_kg output; mdot_cons_kgs input; dt_s input; SOC_H2 output; P_tank_bar output
function [m_H2_kg, SOC_H2, P_tank_bar] = tank_dynamics(mdot_prod_kgs, mdot_cons_kgs, dt_s)
%#codegen
% Signal-level H2 tank (NO electrical). Mass-balance integrator + SOC + Z-
% corrected real-gas pressure. See build_h2tank.m T2-T4.
m0 = 500;  m_cap = 1000;  m_min = 50;  m_max = 950;
Z = 1.2;  Rgas = 8.314;  TK = 298.15;  MH2 = 0.002016;  Vtank = 42.156787;
    persistent m
    if isempty(m), m = m0; end

    % ── mass balance (T2): production ADDS, consumption REMOVES.
    %    Both inputs arrive as +kg/s (IO_CONTRACTS §1.1) → subtract cons.
    m = m + (mdot_prod_kgs - mdot_cons_kgs)*dt_s;

    % ── SOC limits [0.05,0.95] → m∈[m_min,m_max] (T3, Rule 7). The clamp is
    %    the anti-windup FREEZE: at a rail the state holds, so a full tank
    %    cannot overfill nor an empty tank go negative (physical constraint).
    if m > m_max, m = m_max; end
    if m < m_min, m = m_min; end

    % ── outputs
    m_H2_kg = m;
    SOC_H2  = m / m_cap;                      % bounded [0.05, 0.95]

    % ── real-gas pressure (T4): P = Z·m·R·T/(M·V). H2 @350 bar is NOT ideal —
    %    Z≈1.2 (small molecule, repulsive regime) → real P is ~20% above the
    %    ideal-gas value for the same mass. Vtank sized so m_cap → P_max.
    P_tank_bar = Z * m * Rgas * TK / (MH2 * Vtank) / 1e5;
end

== stateflow chart microgrid_case5/EMS/EMS_Chart ==
  settings: updateMethod=DISCRETE  sampleTime=0.1
  state GRID_CONNECTED
    entry:
    state_id = 1;
    during:
    % GRID PRIORITY LADDER. The PV+Wind on the DC bus are a resource to USE (the
    % grid independently covers the AC load). Order: (1) charge battery, (2) run
    % electrolyzer, (3) whatever is left raises V_dc and the VSC DC-link droop
    % exports it to the grid (build_vsc, part A — no EMS command needed).
    Pnet = P_pv + P_wind - P_load;     % kept for reference only
    Prenew = P_pv + P_wind;            % DC generation to absorb / store / export
    % priority 1: charge the battery with renewables until SOC reaches EL_on
    Pchg = 0;
    if SOC_ESS < EL_on
    Pchg = min(Pessmax, Prenew);
    end
    Pref_ess = -Pchg;                  % - = charge
    % priority 2: electrolyzer absorbs the renewable BEYOND the battery, once the
    % battery is full enough (hysteresis) and the tank has room
    if SOC_ESS >= EL_on && SOC_H2 < H2_full
    el_on = 1;
    end
    if SOC_ESS <= EL_off || SOC_H2 >= H2_full
    el_on = 0;
    end
    if el_on > 0.5
    Pcmd_elec = min(Pelmax, max(Pelmin, Prenew - Pchg));
    else
    Pcmd_elec = 0;
    end
    % priority 3: surplus beyond battery+EL -> VSC exports (V_dc droop, part A).
    Pcmd_fc = 0;                       % grid mode: FC off, preserve H2
    % EMERGENCY debounce (M10): count consecutive ticks with |Δf|≥df_em so a single
    % 1-sample PLL/measurement spike at a load-switch instant cannot trip EMERGENCY;
    % a genuine excursion persists and still trips after N_emerg ticks (definite-time).
    if abs(f_meas - f0) >= df_em
    emerg_cnt = emerg_cnt + 1;
    else
    emerg_cnt = 0;
    end
  state ISLAND_TRANSITION
    entry:
    state_id = 2;
    t_island = 0;
    pnet_lpf = P_pv + P_wind - P_load; % seed the LPF for ISLAND_STABLE
    f_prev = f_meas;   % prime the RoCoF backward difference
    rocof  = 999;      % sentinel: block the settle-guard until a REAL df/dt exists
    during:
    t_island = t_island + dt;
    rocof  = (f_meas - f_prev) / dt;   % RoCoF estimate [Hz/s] (settling detector)
    f_prev = f_meas;                   % update backward diff for next cycle
    Pcmd_elec = 0;     % FREEZE hydrogen (electrolyzer off)
    Pref_ess = 0;      % let the VSC battery droop take over; EMS does not fight
    el_on = 0;
    % Pcmd_fc is intentionally NOT written here -> the Stateflow output HOLDS its
    % last commanded value (FC frozen; tau_FC cannot follow the transient anyway).
    % EMERGENCY debounce (M10): reject a single-sample PLL spike at the islanding
    % instant; a genuine excursion still trips after N_emerg consecutive ticks.
    if abs(f_meas - f0) >= df_em
    emerg_cnt = emerg_cnt + 1;
    else
    emerg_cnt = 0;
    end
  state EMERGENCY
    entry:
    state_id = 4;
    emerg_cnt = 0;    % M10: clear the debounce counter on entry so a STALE count
    % (frozen while in EMERGENCY, which does not update it) cannot
    % re-fire GRID/STABLE->EMERGENCY on exit -> no GRID<->EMERG chatter.
    % Re-entry then needs N_emerg FRESH consecutive over-threshold ticks.
    during:
    df = f_meas - f0;
    if df < 0
    % under-frequency (deficit): all generation to the rail, electrolyzer OFF
    Pref_ess = Pessmax;
    Pcmd_fc = Pfcmax;
    Pcmd_elec = 0;
    fc_on = 1; el_on = 0;
    else
    % over-frequency (surplus): absorb hard, FC off (M6 sign-aware dual)
    Pref_ess = -Pessmax;
    Pcmd_elec = Pelmax;
    Pcmd_fc = 0;
    el_on = 1; fc_on = 0;
    end
  state ISLAND_STABLE
    entry:
    state_id = 3;
    during:
    Pnet = P_pv + P_wind - P_load;
    % TIME-SCALE SPLIT: slow (LPF) part -> hydrogen, fast residual -> battery
    pnet_lpf = pnet_lpf + (Pnet - pnet_lpf) * dt / tau_h2;
    % electrolyzer hysteresis (absorb sustained surplus)
    if SOC_ESS >= EL_on && pnet_lpf > 0 && SOC_H2 < H2_full
    el_on = 1;
    end
    if SOC_ESS <= EL_off || pnet_lpf <= 0 || SOC_H2 >= H2_full
    el_on = 0;
    end
    % fuel-cell hysteresis (M3) — engage H2 on a SUSTAINED deficit the battery
    % cannot hold alone (A6/R4). Trigger on EITHER a drained battery (SOC low) OR
    % the slow deficit reaching the battery working ceiling FCpdon (heavy island).
    if (SOC_ESS <= FC_on || (-pnet_lpf) >= FCpdon) && pnet_lpf < 0 && SOC_H2 > H2_empty
    fc_on = 1;
    end
    % OFF only when BOTH drain reasons are clearly cleared (SOC recovered AND deficit
    % below the FCpdoff deadband), or there is no deficit, or the tank is empty.
    if (SOC_ESS >= FC_off && (-pnet_lpf) <= FCpdoff) || pnet_lpf >= 0 || SOC_H2 <= H2_empty
    fc_on = 0;
    end
    if el_on > 0.5
    Pcmd_elec = min(Pelmax, max(Pelmin, pnet_lpf));
    else
    Pcmd_elec = 0;
    end
    if fc_on > 0.5
    if SOC_ESS <= FC_on
    % drained battery -> FC carries the whole slow deficit (rest the battery)
    Pcmd_fc = min(Pfcmax, max(Pfcmin, -pnet_lpf));
    else
    % healthy battery carries up to its working ceiling FCpdon; FC tops up ONLY
    % the excess (H2 = last resort). Battery then stays off its ±Pessmax ceiling.
    Pcmd_fc = min(Pfcmax, max(Pfcmin, (-pnet_lpf) - FCpdon));
    end
    else
    Pcmd_fc = 0;
    end
    % battery holds the remaining balance (gets the fast residual)
    Pref_ess = max(-Pessmax, min(Pessmax, -Pnet + Pcmd_elec - Pcmd_fc));
    % EMERGENCY debounce (M10): a single-sample |Δf| spike (PLL glitch at a load step)
    % must NOT trip EMERGENCY; require N_emerg consecutive ticks (definite-time).
    if abs(f_meas - f0) >= df_em
    emerg_cnt = emerg_cnt + 1;
    else
    emerg_cnt = 0;
    end
  (default) -> GRID_CONNECTED
  ISLAND_TRANSITION -> EMERGENCY [order 1] : [emerg_cnt >= N_emerg]
  GRID_CONNECTED -> ISLAND_TRANSITION [order 2] : [CB1 < 0.5]
  ISLAND_TRANSITION -> GRID_CONNECTED [order 2] : [CB1 >= 0.5]
  GRID_CONNECTED -> EMERGENCY [order 1] : [emerg_cnt >= N_emerg]
  ISLAND_STABLE -> GRID_CONNECTED [order 2] : [CB1 >= 0.5]
  EMERGENCY -> GRID_CONNECTED [order 1] : [abs(f_meas - f0) <= df_cl && CB1 >= 0.5]
  ISLAND_TRANSITION -> ISLAND_STABLE [order 3] : [abs(rocof) < rocof_se || t_island > t_tmax]
  ISLAND_STABLE -> EMERGENCY [order 1] : [emerg_cnt >= N_emerg]
  EMERGENCY -> ISLAND_STABLE [order 2] : [abs(f_meas - f0) <= df_cl && CB1 < 0.5]
  data: f_meas input; SOC_ESS input; SOC_H2 input; CB1 input; P_pv input; P_wind input; P_load input; dt input; Pref_ess output; Pcmd_elec output; Pcmd_fc output; state_id output; el_on local =0; fc_on local =0; t_island local =0; pnet_lpf local =0; Pnet local =0; df local =0; Prenew local =0; Pchg local =0; f_prev local =0; rocof local =0; emerg_cnt local =0; f0 constant double =50; EL_on constant double =0.8; EL_off constant double =0.75; FC_on constant double =0.25; FC_off constant double =0.3; H2_full constant double =0.95; H2_empty constant double =0.05; Pelmin constant double =5; Pelmax constant double =40; Pfcmin constant double =2; Pfcmax constant double =30; Pessmax constant double =80; FCpdon constant double =72; FCpdoff constant double =64; df_em constant double =1.5; df_cl constant double =0.8; rocof_se constant double =0.2; t_tmax constant double =1.5; tau_h2 constant double =20; N_emerg constant double =2

== matlab function microgrid_case5/TransmissionNetwork/SM_Bus1/Pe_calc ==
  data: V_abc input; P_elec_MW output; I_abc input
function P_elec_MW = Pe_calc(V_abc, I_abc)
%#codegen
% Instantaneous 3-phase electrical power at the machine terminal [MW].
    P_W       = V_abc(1)*I_abc(1) + V_abc(2)*I_abc(2) + V_abc(3)*I_abc(3);
    P_elec_MW = P_W / 1e6;
end

== matlab function microgrid_case5/TransmissionNetwork/SM_Bus1/Swing_Eq ==
  data: P_mech_MW input; domega_pu_dt output; P_elec_MW input; omega_pu input; H_sec input; D_pu input; S_base_MW input
function domega_pu_dt = swing_eq(P_mech_MW, P_elec_MW, omega_pu, H_sec, D_pu, S_base_MW)
%#codegen
% Classical swing equation, per-unit, Rule-2 form 1/(2H*s + D).
% Per-unit base = machine MVA rating (Rule 3, single-machine row).
    dP_pu        = (P_mech_MW - P_elec_MW) / S_base_MW;
    dOmega_pu    = omega_pu - 1.0;
    domega_pu_dt = (dP_pu - D_pu * dOmega_pu) / (2 * H_sec);
end

== matlab function microgrid_case5/TransmissionNetwork/SM_Bus3/Swing_Eq ==
  data: P_mech_MW input; domega_pu_dt output; P_elec_MW input; omega_pu input; H_sec input; D_pu input; S_base_MW input
function domega_pu_dt = swing_eq(P_mech_MW, P_elec_MW, omega_pu, H_sec, D_pu, S_base_MW)
%#codegen
% Classical swing equation, per-unit, Rule-2 form 1/(2H*s + D).
% Per-unit base = machine MVA rating (Rule 3, single-machine row).
    dP_pu        = (P_mech_MW - P_elec_MW) / S_base_MW;
    dOmega_pu    = omega_pu - 1.0;
    domega_pu_dt = (dP_pu - D_pu * dOmega_pu) / (2 * H_sec);
end

== matlab function microgrid_case5/TransmissionNetwork/SM_Bus3/Pe_calc ==
  data: V_abc input; P_elec_MW output; I_abc input
function P_elec_MW = Pe_calc(V_abc, I_abc)
%#codegen
% Instantaneous 3-phase electrical power at the machine terminal [MW].
    P_W       = V_abc(1)*I_abc(1) + V_abc(2)*I_abc(2) + V_abc(3)*I_abc(3);
    P_elec_MW = P_W / 1e6;
end

== matlab function microgrid_case5/TransmissionNetwork/SM_Bus5/Swing_Eq ==
  data: P_mech_MW input; domega_pu_dt output; P_elec_MW input; omega_pu input; H_sec input; D_pu input; S_base_MW input
function domega_pu_dt = swing_eq(P_mech_MW, P_elec_MW, omega_pu, H_sec, D_pu, S_base_MW)
%#codegen
% Classical swing equation, per-unit, Rule-2 form 1/(2H*s + D).
% Per-unit base = machine MVA rating (Rule 3, single-machine row).
    dP_pu        = (P_mech_MW - P_elec_MW) / S_base_MW;
    dOmega_pu    = omega_pu - 1.0;
    domega_pu_dt = (dP_pu - D_pu * dOmega_pu) / (2 * H_sec);
end
